simulink model "model"  (R2025b)
settings: Solver=ode4  StartTime=0.0  StopTime=p.stop  FixedStep=p.ts  RelTol=1e-3
values from neighbouring files (symbols this model uses):
  p = par    [pins_init.m]    (also in run.m)
libraries: slpidlib x3
settings Model: Creator=Lemon  LastModifiedBy=Lemon

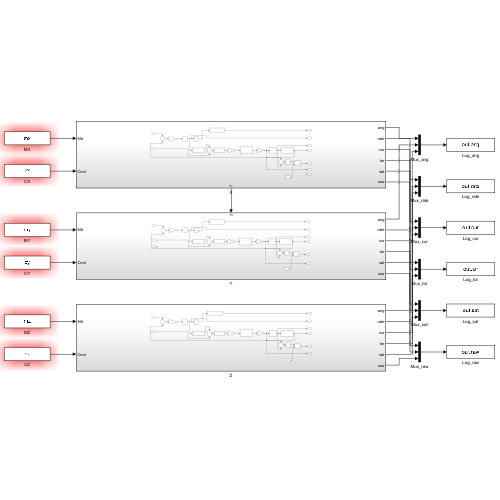
[thumbnail: Simulink's stored preview of the top-level diagram]
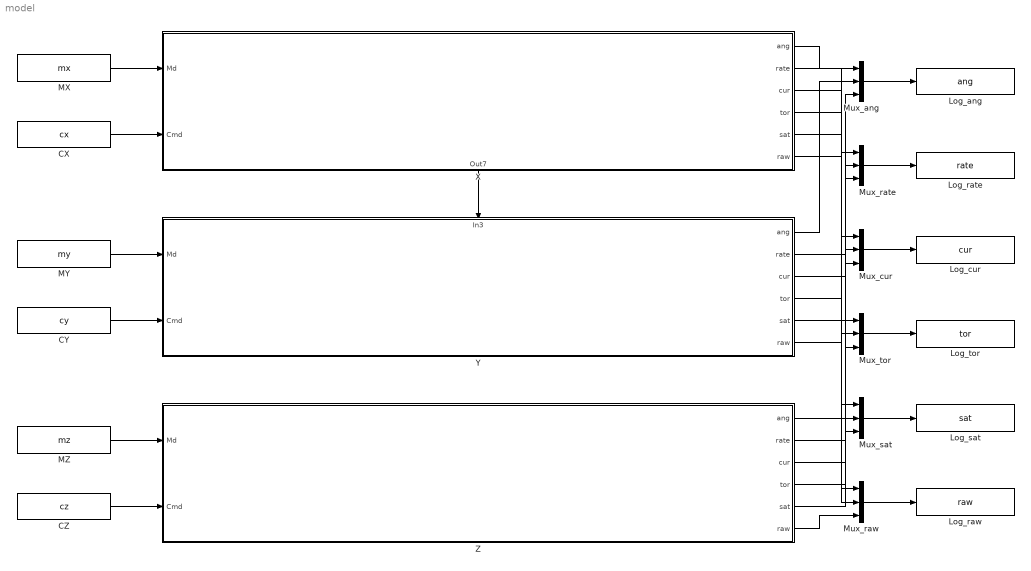
== system model ==
  CX : FromWorkspace  VariableName=cx
  CY : FromWorkspace  VariableName=cy
  CZ : FromWorkspace  VariableName=cz
  Log_ang : ToWorkspace  VariableName=ang  SaveFormat=Timeseries  SampleTime=-1
  Log_cur : ToWorkspace  VariableName=cur  SaveFormat=Timeseries  SampleTime=-1
  Log_rate : ToWorkspace  VariableName=rate  SaveFormat=Timeseries  SampleTime=-1
  Log_raw : ToWorkspace  VariableName=raw  SaveFormat=Timeseries  SampleTime=-1
  Log_sat : ToWorkspace  VariableName=sat  SaveFormat=Timeseries  SampleTime=-1
  Log_tor : ToWorkspace  VariableName=tor  SaveFormat=Timeseries  SampleTime=-1
  MX : FromWorkspace  VariableName=mx
  MY : FromWorkspace  VariableName=my
  MZ : FromWorkspace  VariableName=mz
  Mux_ang : Mux  Inputs=3
  Mux_cur : Mux  Inputs=3
  Mux_rate : Mux  Inputs=3
  Mux_raw : Mux  Inputs=3
  Mux_sat : Mux  Inputs=3
  Mux_tor : Mux  Inputs=3
  X : Subsystem
      settings: PortSchema="{\"entries\":[{\"content\":{\"sides\":[{\"content\":{\"connectorIds\":[\"In1\",\"In2\"]},\"type\":\"ConnectorPlacement.EquallySpacedRectSide\",\"uuid\":\"3dd46c86-2ae8-43e5-bace-620eeb004164\"},{\"content\":{\"connectorIds\":[\"Out1\",\"Out2\",\"Out3\",\"Out4\",\"Out5\",\"Out6\"],\"side\":\"RIGHT\"},\"type\":\"ConnectorPlacement.EquallySpacedRectSide\",\"uuid\":\"82ae68b5-50c6-4e9f-bbdc-800d1ee11391\"},{\"content\":{\"side\":\"TOP\"},\"type\":\"ConnectorPlacement.EquallySpacedRectSide\",\"uuid\":\"ed3ca54a-0448-467b-8892-4752060b7b4e\"},{\"content\":{\"connectorIds\":[\"Out7\"],\"side\":\"BOTTOM\"},\"type\":\"ConnectorPlacement.EquallySpacedRectSide\",\"uuid\":\"bc598dc7-14f7-4a92-83b0-1b130e0c9058\"}]},\"type\":\"ConnectorPlacement.EquallySpacedConnector\",\"uuid\":\"1105bed5-75d5-427c-8f66-c6891da92244\"}],\"packageUris\":[\"http://schema.mathworks.com/mf0/Connector/R2020b\"],\"version\":\"1.0\"}"
  Y : Subsystem
      settings: PortSchema="{\"entries\":[{\"content\":{\"sides\":[{\"content\":{\"connectorIds\":[\"In1\",\"In2\"]},\"type\":\"ConnectorPlacement.EquallySpacedRectSide\",\"uuid\":\"3dd46c86-2ae8-43e5-bace-620eeb004164\"},{\"content\":{\"connectorIds\":[\"Out1\",\"Out2\",\"Out3\",\"Out4\",\"Out5\",\"Out6\"],\"side\":\"RIGHT\"},\"type\":\"ConnectorPlacement.EquallySpacedRectSide\",\"uuid\":\"82ae68b5-50c6-4e9f-bbdc-800d1ee11391\"},{\"content\":{\"connectorIds\":[\"In3\"],\"side\":\"TOP\"},\"type\":\"ConnectorPlacement.EquallySpacedRectSide\",\"uuid\":\"ed3ca54a-0448-467b-8892-4752060b7b4e\"}]},\"type\":\"ConnectorPlacement.EquallySpacedConnector\",\"uuid\":\"1105bed5-75d5-427c-8f66-c6891da92244\"}],\"packageUris\":[\"http://schema.mathworks.com/mf0/Connector/R2020b\"],\"version\":\"1.0\"}"
  Z : Subsystem
  wires:
  MX/1 -> X/1(Md)
  CX/1 -> X/2(Cmd)
  MY/1 -> Y/1(Md)
  CY/1 -> Y/2(Cmd)
  MZ/1 -> Z/1(Md)
  CZ/1 -> Z/2(Cmd)
  X/1(ang) -> Mux_ang/1
  Y/1(ang) -> Mux_ang/2
  Z/1(ang) -> Mux_ang/3
  Mux_ang/1 -> Log_ang/1
  X/2(rate) -> Mux_rate/1
  Y/2(rate) -> Mux_rate/2
  Z/2(rate) -> Mux_rate/3
  Mux_rate/1 -> Log_rate/1
  X/3(cur) -> Mux_cur/1
  Y/3(cur) -> Mux_cur/2
  Z/3(cur) -> Mux_cur/3
  Mux_cur/1 -> Log_cur/1
  X/4(tor) -> Mux_tor/1
  Y/4(tor) -> Mux_tor/2
  Z/4(tor) -> Mux_tor/3
  Mux_tor/1 -> Log_tor/1
  X/5(sat) -> Mux_sat/1
  Y/5(sat) -> Mux_sat/2
  Z/5(sat) -> Mux_sat/3
  Mux_sat/1 -> Log_sat/1
  X/6(raw) -> Mux_raw/1
  Y/6(raw) -> Mux_raw/2
  Z/6(raw) -> Mux_raw/3
  Mux_raw/1 -> Log_raw/1
  X/7(Out7) -> Y/3(In3)

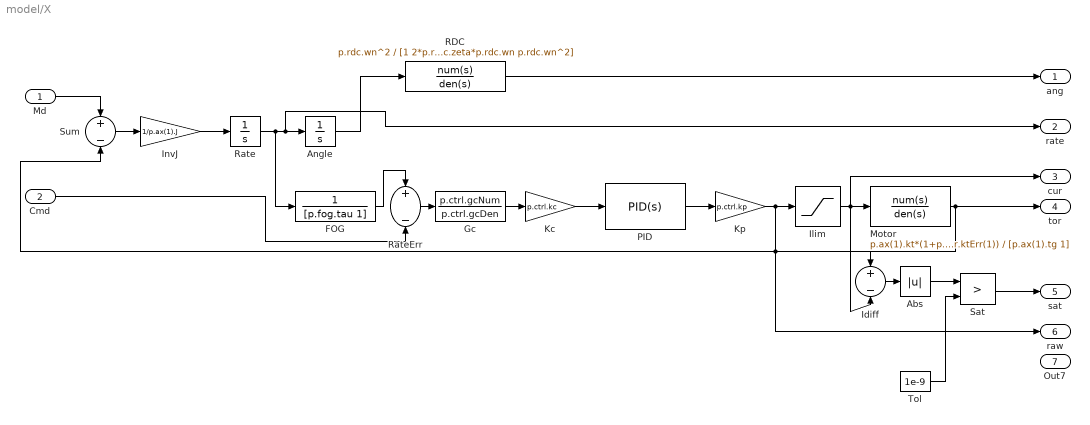
== system model/X ==
  Md : Inport
  Cmd : Inport  Port=2
  Abs : Abs  SaturateOnIntegerOverflow=off
  Angle : Integrator
  FOG : TransferFcn  Numerator=1  Denominator=[p.fog.tau 1]
  Gc : TransferFcn  Numerator=p.ctrl.gcNum  Denominator=p.ctrl.gcDen
  Idiff : Sum  Inputs=+-
  Ilim : Saturate  UpperLimit=p.motor.iMax(1)  LowerLimit=-p.motor.iMax(1)
  InvJ : Gain  Gain=1/p.ax(1).J
  Kc : Gain  Gain=p.ctrl.kc
  Kp : Gain  Gain=p.ctrl.kp
  Motor : TransferFcn  Numerator=p.ax(1).kt*(1+p.motor.ktErr(1))  Denominator=[p.ax(1).tg 1]
  PID : slpidlib/PID Controller  Controller=PID  Form=Parallel  TimeDomain=Continuous-time  UseExternalTs=off  SampleTime=-1  IntegratorMethod=Forward Euler  FilterMethod=Forward Euler  ControllerParametersSource=internal  P=p.ctrl.pid(1)  I=p.ctrl.pid(2)  UseKiTs=off  D=p.ctrl.pid(3)  UseExternalDerivativeSource=off  N=p.ctrl.n  UseFilter=on  TunerSelectOption=Transfer Function Based (PID Tuner App)  InitialConditionSource=internal  InitialConditionForIntegrator=0  InitialConditionForFilter=0  DifferentiatorICPrevScaledInput=0  ExternalReset=none  TrackingMode=off  Kt=1  LimitOutput=off  SatLimitsSource=internal  UpperSaturationLimit=inf  LowerSaturationLimit=-inf  LinearizeAsGain=on  AntiWindupMode=none  Kb=1  LimitIntegrator=off  UpperIntegratorSaturationLimit=inf  LowerIntegratorSaturationLimit=-inf  POutMin=[]  POutMax=[]  IOutMin=[]  IOutMax=[]  DOutMin=[]  DOutMax=[]  NOutMin=[]  NOutMax=[]  SumOutMin=[]  SumOutMax=[]  SaturationOutMin=[]  SaturationOutMax=[]  PParamMin=[]  PParamMax=[]  IParamMin=[]  IParamMax=[]  DParamMin=[]  DParamMax=[]  NParamMin=[]  NParamMax=[]  KbParamMin=[]  KbParamMax=[]  KtParamMin=[]  KtParamMax=[]  KbOutMin=[]  KbOutMax=[]  KtOutMin=[]  KtOutMax=[]  IntegratorOutMin=[]  IntegratorOutMax=[]  FilterOutMin=[]  FilterOutMax=[]  SumI1OutMin=[]  SumI1OutMax=[]  SumI2OutMin=[]  SumI2OutMax=[]  SumI3OutMin=[]  SumI3OutMax=[]  SumI4OutMin=[]  SumI4OutMax=[]  SumDOutMin=[]  SumDOutMax=[]  DifferentiatorOutMin=[]  DifferentiatorOutMax=[]  FilterDiffOutCoefMin=[]  FilterDiffOutCoefMax=[]  ReciprocalOutMin=[]  ReciprocalOutMax=[]  SumDenOutMin=[]  SumDenOutMax=[]  SumNumOutMin=[]  SumNumOutMax=[]  DivideOutMin=[]  DivideOutMax=[]  UdiffTsProdOutMin=[]  UdiffTsProdOutMax=[]  NTsProdOutMin=[]  NTsProdOutMax=[]  UintegralTsProdOutMin=[]  UintegralTsProdOutMax=[]  UngainTsProdOutMin=[]  UngainTsProdOutMax=[]  ClampingZeroOutDataTypeStr=Inherit: Inherit via back propagation  ClampingZeroOutMin=[]  ClampingZeroOutMax=[]  FilterDenConstantOutDataTypeStr=Inherit: Inherit via back propagation  FilterDenConstantOutMin=[]  FilterDenConstantOutMax=[]  PCopyOutDataTypeStr=Inherit: Inherit via back propagation  PCopyOutMin=[]  PCopyOutMax=[]  NCopyOutDataTypeStr=Inherit: Inherit via back propagation  NCopyOutMin=[]  NCopyOutMax=[]  IntegratorContinuousStateAttributes=''  IntegratorStateMustResolveToSignalObject=off  IntegratorRTWStateStorageClass=Auto  FilterContinuousStateAttributes=''  FilterStateMustResolveToSignalObject=off  FilterRTWStateStorageClass=Auto  ParallelPVariant=InternalParameters  IdealPVariant=Disabled  IVariant=InternalParameters  DVariant=InternalParameters  IntegratorVariant=Continuous  SatVariant=Disabled  AWVariant=Passthrough  PCopyVariant=Disabled  TRVariant=Disabled  FdbkBlocksVariant=Forward  IdealPFdbkVariant=Disabled  SatFdbkVariant=Disabled  DerivativeFilterVariant=ContFilter  NVariant=InternalParameters  NCopyVariant=Disabled  FilterICVariant=InternalICsFilter  IntegratorICVariant=InternalICs  ExternalResetVariant=Disabled  TRSumVariant=Passthrough  SumFdbkVariant=Disabled  SumVariant=Sum_PID  TsampFilterVariant=InternalTs  TsampNgainVariant=Passthrough  TsampIntegralVariant=Disabled_SignalSpec  ExternalSaturationOutDataTypeStr=Inherit: Same as second input  DerivativeSourceVariant=ErrorSignal  PreIntVariant=InternalPreInt
  RDC : TransferFcn  Numerator=p.rdc.wn^2  Denominator=[1 2*p.rdc.zeta*p.rdc.wn p.rdc.wn^2]
  Rate : Integrator
  RateErr : Sum  Inputs=+-
  Sat : RelationalOperator  Operator=>  OutDataTypeStr=boolean  RndMeth=Simplest  InputSameDT=off
  Sum : Sum  Inputs=+-
  Tol : Constant  Value=1e-9
  ang : Outport
  rate : Outport  Port=2
  cur : Outport  Port=3
  tor : Outport  Port=4
  sat : Outport  Port=5
  raw : Outport  Port=6
  Out7 : Outport  Port=7
  wires:
  Md/1 -> Sum/1
  Sum/1 -> InvJ/1
  InvJ/1 -> Rate/1
  Rate/1 -> Angle/1, rate/1, FOG/1
  FOG/1 -> RateErr/1
  Cmd/1 -> RateErr/2
  RateErr/1 -> Gc/1
  Gc/1 -> Kc/1
  Kc/1 -> PID/1
  PID/1 -> Kp/1
  Kp/1 -> Idiff/1, raw/1, Ilim/1
  Ilim/1 -> Motor/1, Idiff/2, cur/1
  Motor/1 -> Sum/2, tor/1
  Angle/1 -> RDC/1
  Idiff/1 -> Abs/1
  Abs/1 -> Sat/1
  Tol/1 -> Sat/2
  RDC/1 -> ang/1
  Sat/1 -> sat/1

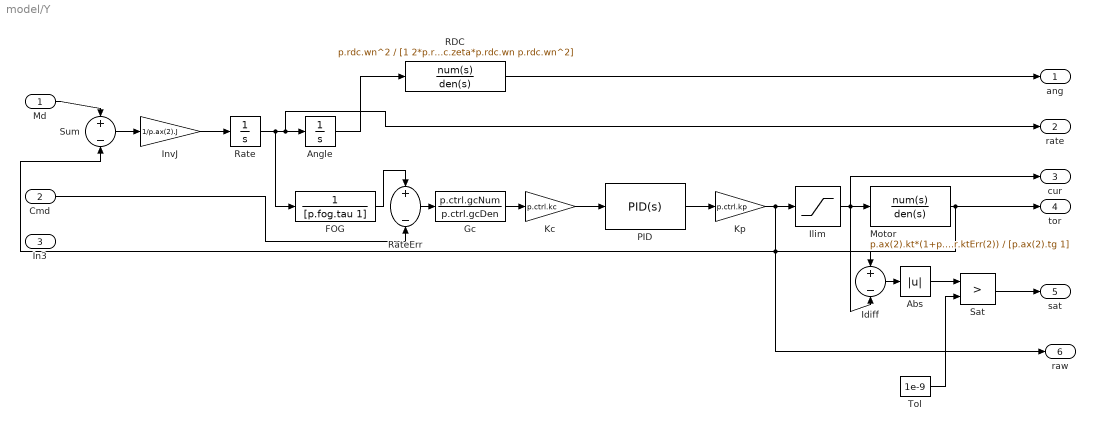
== system model/Y ==
  Md : Inport
  Cmd : Inport  Port=2
  In3 : Inport  Port=3
  Abs : Abs  SaturateOnIntegerOverflow=off
  Angle : Integrator
  FOG : TransferFcn  Numerator=1  Denominator=[p.fog.tau 1]
  Gc : TransferFcn  Numerator=p.ctrl.gcNum  Denominator=p.ctrl.gcDen
  Idiff : Sum  Inputs=+-
  Ilim : Saturate  UpperLimit=p.motor.iMax(2)  LowerLimit=-p.motor.iMax(2)
  InvJ : Gain  Gain=1/p.ax(2).J
  Kc : Gain  Gain=p.ctrl.kc
  Kp : Gain  Gain=p.ctrl.kp
  Motor : TransferFcn  Numerator=p.ax(2).kt*(1+p.motor.ktErr(2))  Denominator=[p.ax(2).tg 1]
  PID : slpidlib/PID Controller  Controller=PID  Form=Parallel  TimeDomain=Continuous-time  UseExternalTs=off  SampleTime=-1  IntegratorMethod=Forward Euler  FilterMethod=Forward Euler  ControllerParametersSource=internal  P=p.ctrl.pid(1)  I=p.ctrl.pid(2)  UseKiTs=off  D=p.ctrl.pid(3)  UseExternalDerivativeSource=off  N=p.ctrl.n  UseFilter=on  TunerSelectOption=Transfer Function Based (PID Tuner App)  InitialConditionSource=internal  InitialConditionForIntegrator=0  InitialConditionForFilter=0  DifferentiatorICPrevScaledInput=0  ExternalReset=none  TrackingMode=off  Kt=1  LimitOutput=off  SatLimitsSource=internal  UpperSaturationLimit=inf  LowerSaturationLimit=-inf  LinearizeAsGain=on  AntiWindupMode=none  Kb=1  LimitIntegrator=off  UpperIntegratorSaturationLimit=inf  LowerIntegratorSaturationLimit=-inf  POutMin=[]  POutMax=[]  IOutMin=[]  IOutMax=[]  DOutMin=[]  DOutMax=[]  NOutMin=[]  NOutMax=[]  SumOutMin=[]  SumOutMax=[]  SaturationOutMin=[]  SaturationOutMax=[]  PParamMin=[]  PParamMax=[]  IParamMin=[]  IParamMax=[]  DParamMin=[]  DParamMax=[]  NParamMin=[]  NParamMax=[]  KbParamMin=[]  KbParamMax=[]  KtParamMin=[]  KtParamMax=[]  KbOutMin=[]  KbOutMax=[]  KtOutMin=[]  KtOutMax=[]  IntegratorOutMin=[]  IntegratorOutMax=[]  FilterOutMin=[]  FilterOutMax=[]  SumI1OutMin=[]  SumI1OutMax=[]  SumI2OutMin=[]  SumI2OutMax=[]  SumI3OutMin=[]  SumI3OutMax=[]  SumI4OutMin=[]  SumI4OutMax=[]  SumDOutMin=[]  SumDOutMax=[]  DifferentiatorOutMin=[]  DifferentiatorOutMax=[]  FilterDiffOutCoefMin=[]  FilterDiffOutCoefMax=[]  ReciprocalOutMin=[]  ReciprocalOutMax=[]  SumDenOutMin=[]  SumDenOutMax=[]  SumNumOutMin=[]  SumNumOutMax=[]  DivideOutMin=[]  DivideOutMax=[]  UdiffTsProdOutMin=[]  UdiffTsProdOutMax=[]  NTsProdOutMin=[]  NTsProdOutMax=[]  UintegralTsProdOutMin=[]  UintegralTsProdOutMax=[]  UngainTsProdOutMin=[]  UngainTsProdOutMax=[]  ClampingZeroOutDataTypeStr=Inherit: Inherit via back propagation  ClampingZeroOutMin=[]  ClampingZeroOutMax=[]  FilterDenConstantOutDataTypeStr=Inherit: Inherit via back propagation  FilterDenConstantOutMin=[]  FilterDenConstantOutMax=[]  PCopyOutDataTypeStr=Inherit: Inherit via back propagation  PCopyOutMin=[]  PCopyOutMax=[]  NCopyOutDataTypeStr=Inherit: Inherit via back propagation  NCopyOutMin=[]  NCopyOutMax=[]  IntegratorContinuousStateAttributes=''  IntegratorStateMustResolveToSignalObject=off  IntegratorRTWStateStorageClass=Auto  FilterContinuousStateAttributes=''  FilterStateMustResolveToSignalObject=off  FilterRTWStateStorageClass=Auto  ParallelPVariant=InternalParameters  IdealPVariant=Disabled  IVariant=InternalParameters  DVariant=InternalParameters  IntegratorVariant=Continuous  SatVariant=Disabled  AWVariant=Passthrough  PCopyVariant=Disabled  TRVariant=Disabled  FdbkBlocksVariant=Forward  IdealPFdbkVariant=Disabled  SatFdbkVariant=Disabled  DerivativeFilterVariant=ContFilter  NVariant=InternalParameters  NCopyVariant=Disabled  FilterICVariant=InternalICsFilter  IntegratorICVariant=InternalICs  ExternalResetVariant=Disabled  TRSumVariant=Passthrough  SumFdbkVariant=Disabled  SumVariant=Sum_PID  TsampFilterVariant=InternalTs  TsampNgainVariant=Passthrough  TsampIntegralVariant=Disabled_SignalSpec  ExternalSaturationOutDataTypeStr=Inherit: Same as second input  DerivativeSourceVariant=ErrorSignal  PreIntVariant=InternalPreInt
  RDC : TransferFcn  Numerator=p.rdc.wn^2  Denominator=[1 2*p.rdc.zeta*p.rdc.wn p.rdc.wn^2]
  Rate : Integrator
  RateErr : Sum  Inputs=+-
  Sat : RelationalOperator  Operator=>  OutDataTypeStr=boolean  RndMeth=Simplest  InputSameDT=off
  Sum : Sum  Inputs=+-
  Tol : Constant  Value=1e-9
  ang : Outport
  rate : Outport  Port=2
  cur : Outport  Port=3
  tor : Outport  Port=4
  sat : Outport  Port=5
  raw : Outport  Port=6
  wires:
  Md/1 -> Sum/1
  Sum/1 -> InvJ/1
  InvJ/1 -> Rate/1
  Rate/1 -> Angle/1, rate/1, FOG/1
  FOG/1 -> RateErr/1
  Cmd/1 -> RateErr/2
  RateErr/1 -> Gc/1
  Gc/1 -> Kc/1
  Kc/1 -> PID/1
  PID/1 -> Kp/1
  Kp/1 -> Idiff/1, raw/1, Ilim/1
  Ilim/1 -> Motor/1, Idiff/2, cur/1
  Motor/1 -> Sum/2, tor/1
  Angle/1 -> RDC/1
  Idiff/1 -> Abs/1
  Abs/1 -> Sat/1
  Tol/1 -> Sat/2
  RDC/1 -> ang/1
  Sat/1 -> sat/1

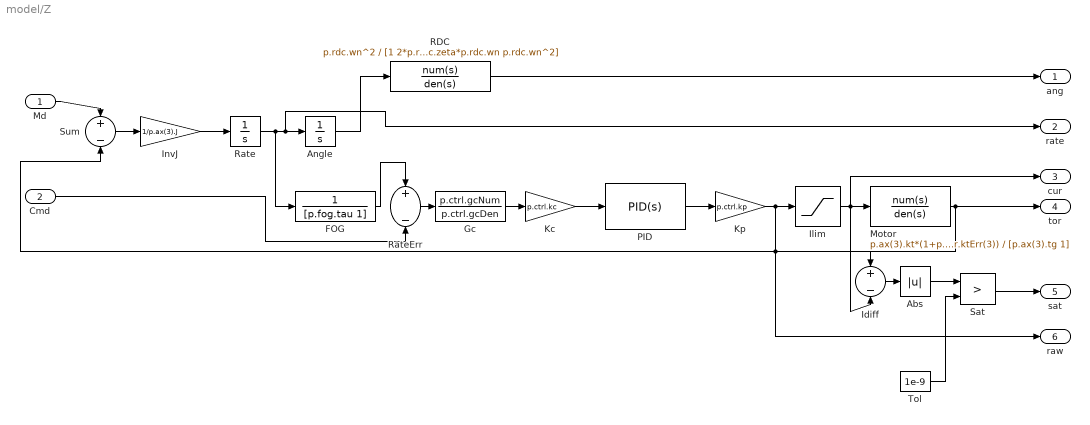
== system model/Z ==
  Md : Inport
  Cmd : Inport  Port=2
  Abs : Abs  SaturateOnIntegerOverflow=off
  Angle : Integrator
  FOG : TransferFcn  Numerator=1  Denominator=[p.fog.tau 1]
  Gc : TransferFcn  Numerator=p.ctrl.gcNum  Denominator=p.ctrl.gcDen
  Idiff : Sum  Inputs=+-
  Ilim : Saturate  UpperLimit=p.motor.iMax(3)  LowerLimit=-p.motor.iMax(3)
  InvJ : Gain  Gain=1/p.ax(3).J
  Kc : Gain  Gain=p.ctrl.kc
  Kp : Gain  Gain=p.ctrl.kp
  Motor : TransferFcn  Numerator=p.ax(3).kt*(1+p.motor.ktErr(3))  Denominator=[p.ax(3).tg 1]
  PID : slpidlib/PID Controller  Controller=PID  Form=Parallel  TimeDomain=Continuous-time  UseExternalTs=off  SampleTime=-1  IntegratorMethod=Forward Euler  FilterMethod=Forward Euler  ControllerParametersSource=internal  P=p.ctrl.pid(1)  I=p.ctrl.pid(2)  UseKiTs=off  D=p.ctrl.pid(3)  UseExternalDerivativeSource=off  N=p.ctrl.n  UseFilter=on  TunerSelectOption=Transfer Function Based (PID Tuner App)  InitialConditionSource=internal  InitialConditionForIntegrator=0  InitialConditionForFilter=0  DifferentiatorICPrevScaledInput=0  ExternalReset=none  TrackingMode=off  Kt=1  LimitOutput=off  SatLimitsSource=internal  UpperSaturationLimit=inf  LowerSaturationLimit=-inf  LinearizeAsGain=on  AntiWindupMode=none  Kb=1  LimitIntegrator=off  UpperIntegratorSaturationLimit=inf  LowerIntegratorSaturationLimit=-inf  POutMin=[]  POutMax=[]  IOutMin=[]  IOutMax=[]  DOutMin=[]  DOutMax=[]  NOutMin=[]  NOutMax=[]  SumOutMin=[]  SumOutMax=[]  SaturationOutMin=[]  SaturationOutMax=[]  PParamMin=[]  PParamMax=[]  IParamMin=[]  IParamMax=[]  DParamMin=[]  DParamMax=[]  NParamMin=[]  NParamMax=[]  KbParamMin=[]  KbParamMax=[]  KtParamMin=[]  KtParamMax=[]  KbOutMin=[]  KbOutMax=[]  KtOutMin=[]  KtOutMax=[]  IntegratorOutMin=[]  IntegratorOutMax=[]  FilterOutMin=[]  FilterOutMax=[]  SumI1OutMin=[]  SumI1OutMax=[]  SumI2OutMin=[]  SumI2OutMax=[]  SumI3OutMin=[]  SumI3OutMax=[]  SumI4OutMin=[]  SumI4OutMax=[]  SumDOutMin=[]  SumDOutMax=[]  DifferentiatorOutMin=[]  DifferentiatorOutMax=[]  FilterDiffOutCoefMin=[]  FilterDiffOutCoefMax=[]  ReciprocalOutMin=[]  ReciprocalOutMax=[]  SumDenOutMin=[]  SumDenOutMax=[]  SumNumOutMin=[]  SumNumOutMax=[]  DivideOutMin=[]  DivideOutMax=[]  UdiffTsProdOutMin=[]  UdiffTsProdOutMax=[]  NTsProdOutMin=[]  NTsProdOutMax=[]  UintegralTsProdOutMin=[]  UintegralTsProdOutMax=[]  UngainTsProdOutMin=[]  UngainTsProdOutMax=[]  ClampingZeroOutDataTypeStr=Inherit: Inherit via back propagation  ClampingZeroOutMin=[]  ClampingZeroOutMax=[]  FilterDenConstantOutDataTypeStr=Inherit: Inherit via back propagation  FilterDenConstantOutMin=[]  FilterDenConstantOutMax=[]  PCopyOutDataTypeStr=Inherit: Inherit via back propagation  PCopyOutMin=[]  PCopyOutMax=[]  NCopyOutDataTypeStr=Inherit: Inherit via back propagation  NCopyOutMin=[]  NCopyOutMax=[]  IntegratorContinuousStateAttributes=''  IntegratorStateMustResolveToSignalObject=off  IntegratorRTWStateStorageClass=Auto  FilterContinuousStateAttributes=''  FilterStateMustResolveToSignalObject=off  FilterRTWStateStorageClass=Auto  ParallelPVariant=InternalParameters  IdealPVariant=Disabled  IVariant=InternalParameters  DVariant=InternalParameters  IntegratorVariant=Continuous  SatVariant=Disabled  AWVariant=Passthrough  PCopyVariant=Disabled  TRVariant=Disabled  FdbkBlocksVariant=Forward  IdealPFdbkVariant=Disabled  SatFdbkVariant=Disabled  DerivativeFilterVariant=ContFilter  NVariant=InternalParameters  NCopyVariant=Disabled  FilterICVariant=InternalICsFilter  IntegratorICVariant=InternalICs  ExternalResetVariant=Disabled  TRSumVariant=Passthrough  SumFdbkVariant=Disabled  SumVariant=Sum_PID  TsampFilterVariant=InternalTs  TsampNgainVariant=Passthrough  TsampIntegralVariant=Disabled_SignalSpec  ExternalSaturationOutDataTypeStr=Inherit: Same as second input  DerivativeSourceVariant=ErrorSignal  PreIntVariant=InternalPreInt
  RDC : TransferFcn  Numerator=p.rdc.wn^2  Denominator=[1 2*p.rdc.zeta*p.rdc.wn p.rdc.wn^2]
  Rate : Integrator
  RateErr : Sum  Inputs=+-
  Sat : RelationalOperator  Operator=>  OutDataTypeStr=boolean  RndMeth=Simplest  InputSameDT=off
  Sum : Sum  Inputs=+-
  Tol : Constant  Value=1e-9
  ang : Outport
  rate : Outport  Port=2
  cur : Outport  Port=3
  tor : Outport  Port=4
  sat : Outport  Port=5
  raw : Outport  Port=6
  wires:
  Md/1 -> Sum/1
  Sum/1 -> InvJ/1
  InvJ/1 -> Rate/1
  Rate/1 -> Angle/1, rate/1, FOG/1
  FOG/1 -> RateErr/1
  Cmd/1 -> RateErr/2
  RateErr/1 -> Gc/1
  Gc/1 -> Kc/1
  Kc/1 -> PID/1
  PID/1 -> Kp/1
  Kp/1 -> Idiff/1, raw/1, Ilim/1
  Ilim/1 -> Motor/1, Idiff/2, cur/1
  Motor/1 -> Sum/2, tor/1
  Angle/1 -> RDC/1
  Idiff/1 -> Abs/1
  Abs/1 -> Sat/1
  Tol/1 -> Sat/2
  RDC/1 -> ang/1
  Sat/1 -> sat/1
